simulink model "system"  (R2023a)
settings: Solver=ode15s  StartTime=0.0  StopTime=10.0  MaxStep=1E-3  RelTol=1e-3
libraries: fl_lib x14, nesl_utility x6, slpidlib x1
settings Model: LastModifiedBy=kevin
settings DataIOCC: SaveFormat=Array  ReturnWorkspaceOutputs=off  TimeSaveName=t
settings DebuggingCC: AlgebraicLoopMsg=none  ArtificialAlgebraicLoopMsg=none  MaxConsecutiveZCsMsg=none  ModelReferenceExtraNoncontSigs=none  OperatingPointInterfaceChecksumMismatchMsg=none
settings RTWCC: GPUComputeCapability=5.0

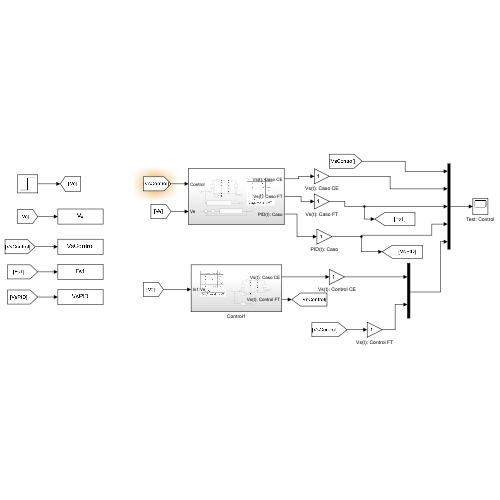
[thumbnail: Simulink's stored preview of the top-level diagram]
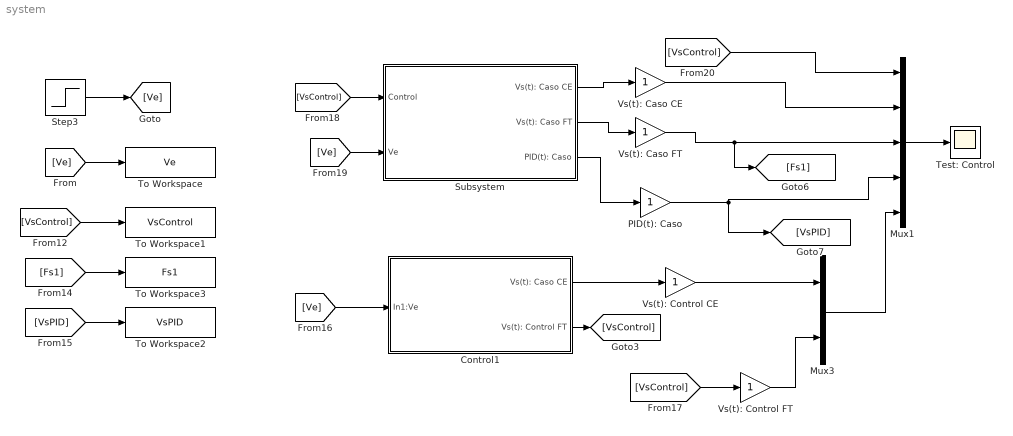
== system system ==
  Control1 : Subsystem
  Mux1 : Mux  Inputs=5
  Mux3 : Mux  Inputs=2
  PID(t): Caso : Gain
  Step3 : Step  Time=0  SampleTime=0
  Subsystem : Subsystem
  Test: Control : Scope
  To Workspace : ToWorkspace  VariableName=Ve  SampleTime=-1
  To Workspace1 : ToWorkspace  VariableName=VsControl  SampleTime=-1
  To Workspace2 : ToWorkspace  VariableName=VsPID  SampleTime=-1
  To Workspace3 : ToWorkspace  VariableName=Fs1  SampleTime=-1
  Vs(t): Caso CE : Gain
  Vs(t): Caso FT : Gain
  Vs(t): Control CE : Gain
  Vs(t): Control FT : Gain
  wires:
  Control1/2(Vs(t): Control FT) -> [VsControl]
  Mux3/1 -> Mux1/5
  Vs(t): Caso CE/1 -> Mux1/2
  Subsystem/3(PID(t): Caso) -> PID(t): Caso/1
  [VsControl] -> Mux1/1
  Mux1/1 -> Test: Control/1
  [Ve] -> Control1/1(In1:Ve)
  [Ve] -> Subsystem/2(Ve)
  [VsControl] -> Subsystem/1(Control)
  Vs(t): Control FT/1 -> Mux3/2
  Subsystem/1(Vs(t): Caso CE) -> Vs(t): Caso CE/1
  PID(t): Caso/1 -> [VsPID], Mux1/4
  [Fs1] -> To Workspace3/1
  [VsControl] -> Vs(t): Control FT/1
  Subsystem/2(Vs(t): Caso FT) -> Vs(t): Caso FT/1
  [VsControl] -> To Workspace1/1
  Control1/1(Vs(t): Caso CE) -> Vs(t): Control CE/1
  Step3/1 -> [Ve]
  Vs(t): Control CE/1 -> Mux3/1
  Vs(t): Caso FT/1 -> [Fs1], Mux1/3
  [Ve] -> To Workspace/1
  [VsPID] -> To Workspace2/1

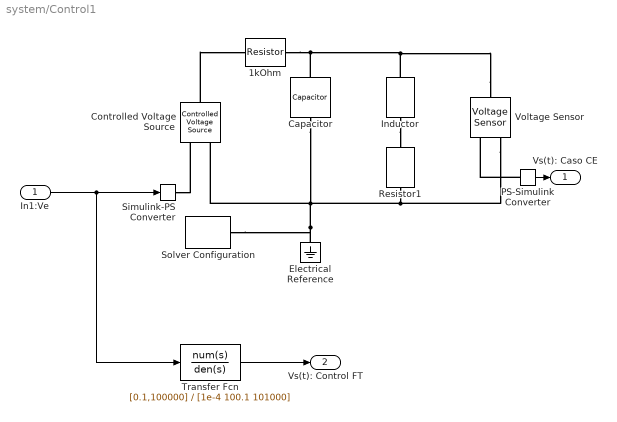
== system system/Control1 ==
  In1:Ve : Inport
  1kOhm : fl_lib/Electrical/Electrical Elements/Resistor  R=1 kOhm  i_specify=off  i_priority=None  i=0 A  i_nominal_specify=off  i_nominal_unit=A  i_nominal_value=1  v_specify=off  v_priority=None  v=0 V  v_nominal_specify=off  v_nominal_unit=V  v_nominal_value=1
  Capacitor : fl_lib/Electrical/Electrical Elements/Capacitor  c=1 uF  r=1e-6 Ohm  g=0 1/Ohm  i_specify=off  i_priority=None  i=0 A  i_nominal_specify=off  i_nominal_unit=A  i_nominal_value=1  v_specify=off  v_priority=None  v=0 V  v_nominal_specify=off  v_nominal_unit=V  v_nominal_value=1  vc_specify=off  vc_priority=High  vc=0 V  vc_nominal_specify=off  vc_nominal_unit=V  vc_nominal_value=1
  Controlled Voltage Source : fl_lib/Electrical/Electrical Sources/Controlled Voltage Source
  Electrical Reference : fl_lib/Electrical/Electrical Elements/Electrical Reference
  Inductor : fl_lib/Electrical/Electrical Elements/Inductor  l=100 mH  r=0 Ohm  g=1e-9 1/Ohm  i_specify=off  i_priority=None  i=0 A  i_nominal_specify=off  i_nominal_unit=A  i_nominal_value=1  v_specify=off  v_priority=None  v=0 V  v_nominal_specify=off  v_nominal_unit=V  v_nominal_value=1  i_L_specify=off  i_L_priority=High  i_L=0 A  i_L_nominal_specify=off  i_L_nominal_unit=A  i_L_nominal_value=1
  PS-Simulink Converter : nesl_utility/PS-Simulink Converter  PhysicalDomain=network_engine_domain  SubClassName=ps_output  LeftPortType=input  RightPortType=output  PseudoPeriodic=off  Frequencies=[]  VectorFormat=inherit  Unit=inherit  AffineConversion=off
  Resistor1 : fl_lib/Electrical/Electrical Elements/Resistor  R=100 kOhm  i_specify=off  i_priority=None  i=0 A  i_nominal_specify=off  i_nominal_unit=A  i_nominal_value=1  v_specify=off  v_priority=None  v=0 V  v_nominal_specify=off  v_nominal_unit=V  v_nominal_value=1
  Simulink-PS Converter : nesl_utility/Simulink-PS Converter  PhysicalDomain=network_engine_domain  SubClassName=ps_input  LeftPortType=input  RightPortType=output  PseudoPeriodic=off  Frequencies=[]  NoiseDistribution=none  NoiseParameters=[]  Unit=1  AffineConversion=off  FilteringAndDerivatives=provide  SimscapeFilterOrder=1  InputFilterTimeConstant=0.001  UdotUserProvided=0
  Solver Configuration : nesl_utility/Solver Configuration  PhysicalDomain=network_engine_domain  SubClassName=solver  LeftPortType=input  RightPortType=generic  Tones=[]  Harmonics=[]  SimulateNoise=off  Profile=off  UseLocalSampling=off  EnableSwitchedLinearOptims=on  FrequencyDomain=off  UseCCode=off  RelTol=0.001  AbsTol=0.001  MinStep=1e-09  ToWorkspace=off  RevertToSquareIcSolve=off  NumHomotopyIterations=100  PhasorMode=off  PhasorModeNumHarmonics=1  ConsistencySolver=NEWTON_XTOL_AFTER_FTOL  IndexReductionMethod=DerivativeReplacement  DoDC=off  ResidualTolerance=1e-09  ConsistencyTolSource=GLOBAL  ConsistencyAbsTol=0.001  ConsistencyRelTol=0.001  ConsistencyTolFactor=0.001  UseLocalSolver=off  LocalSolverChoice=NE_BACKWARD_EULER_ADVANCER  ResolveIndetEquations=on  FunctionEvalNumThread=1  LocalSolverSampleTime=0.001  DoFixedCost=off  MaxNonlinIter=3  MaxModeIter=2  ComputeImpulses=off  ImpulseIterations=2  LinearAlgebra=auto  LinearAlgebraNumThread=0  EquationFormulation=NE_TIME_EF  DelaysMemoryBudget=1024  AutomaticFiltering=on  FilteringTimeConstant=0.001  PartitionStorageMethod=AS_NEEDED  PartitionMemoryBudget=1024  PartitionMethod=ROBUST
  Transfer Fcn : TransferFcn  Numerator=[0.1,100000]  Denominator=[1e-4 100.1 101000]
  Voltage Sensor : fl_lib/Electrical/Electrical Sensors/Voltage Sensor
  Vs(t): Caso CE : Outport
  Vs(t): Control FT : Outport  Port=2
  wires:
  PS-Simulink Converter/1 -> Vs(t): Caso CE/1
  In1:Ve/1 -> Transfer Fcn/1, Simulink-PS Converter/1
  Transfer Fcn/1 -> Vs(t): Control FT/1
  connections:
  Controlled Voltage Source/RConn2 -- Solver Configuration/RConn1 -- Electrical Reference/LConn1 -- Resistor1/LConn1 -- Voltage Sensor/RConn2 -- Capacitor/RConn1
  Voltage Sensor/LConn1 -- 1kOhm/RConn1 -- Capacitor/LConn1 -- Inductor/LConn1
  Inductor/RConn1 -- Resistor1/RConn1
  Simulink-PS Converter/RConn1 -- Controlled Voltage Source/RConn1
  PS-Simulink Converter/LConn1 -- Voltage Sensor/RConn1
  Controlled Voltage Source/LConn1 -- 1kOhm/LConn1

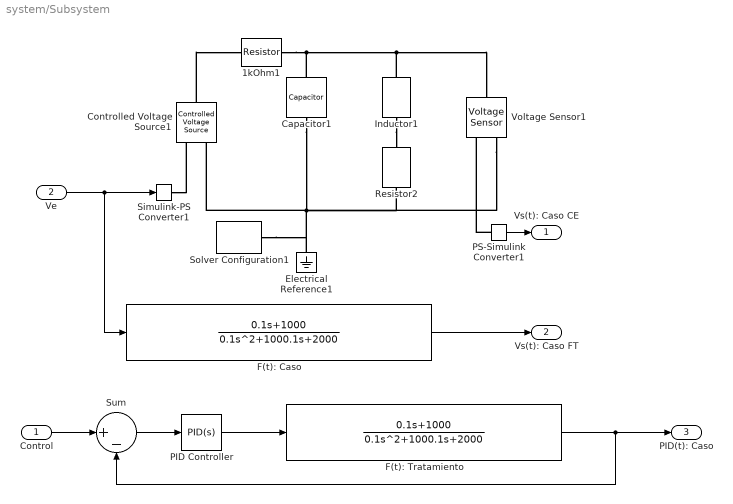
== system system/Subsystem ==
  Control : Inport
  Ve : Inport  Port=2
  1kOhm1 : fl_lib/Electrical/Electrical Elements/Resistor  R=1 kOhm  i_specify=off  i_priority=None  i=0 A  i_nominal_specify=off  i_nominal_unit=A  i_nominal_value=1  v_specify=off  v_priority=None  v=0 V  v_nominal_specify=off  v_nominal_unit=V  v_nominal_value=1
  Capacitor1 : fl_lib/Electrical/Electrical Elements/Capacitor  c=1000 uF  r=1e-6 Ohm  g=0 1/Ohm  i_specify=off  i_priority=None  i=0 A  i_nominal_specify=off  i_nominal_unit=A  i_nominal_value=1  v_specify=off  v_priority=None  v=0 V  v_nominal_specify=off  v_nominal_unit=V  v_nominal_value=1  vc_specify=off  vc_priority=High  vc=0 V  vc_nominal_specify=off  vc_nominal_unit=V  vc_nominal_value=1
  Controlled Voltage Source1 : fl_lib/Electrical/Electrical Sources/Controlled Voltage Source
  Electrical Reference1 : fl_lib/Electrical/Electrical Elements/Electrical Reference
  F(t): Caso : TransferFcn  Numerator=[0.1 1000]  Denominator=[0.1 1000.1 2000]
  F(t): Tratamiento : TransferFcn  Numerator=[0.1 1000]  Denominator=[0.1 1000.1 2000]
  Inductor1 : fl_lib/Electrical/Electrical Elements/Inductor  l=100 mH  r=0 Ohm  g=1e-9 1/Ohm  i_specify=off  i_priority=None  i=0 A  i_nominal_specify=off  i_nominal_unit=A  i_nominal_value=1  v_specify=off  v_priority=None  v=0 V  v_nominal_specify=off  v_nominal_unit=V  v_nominal_value=1  i_L_specify=off  i_L_priority=High  i_L=0 A  i_L_nominal_specify=off  i_L_nominal_unit=A  i_L_nominal_value=1
  PID Controller : slpidlib/PID Controller  Controller=PID  Form=Parallel  TimeDomain=Continuous-time  UseExternalTs=off  SampleTime=-1  IntegratorMethod=Forward Euler  FilterMethod=Forward Euler  ControllerParametersSource=internal  P=400  I=1200  UseKiTs=off  D=0.5  N=2000  UseFilter=on  TunerSelectOption=Transfer Function Based (PID Tuner App)  InitialConditionSource=internal  InitialConditionForIntegrator=0  InitialConditionForFilter=0  DifferentiatorICPrevScaledInput=0  ExternalReset=none  TrackingMode=off  Kt=1  LimitOutput=off  SatLimitsSource=internal  UpperSaturationLimit=inf  LowerSaturationLimit=-inf  LinearizeAsGain=on  AntiWindupMode=none  Kb=1  LimitIntegrator=off  UpperIntegratorSaturationLimit=inf  LowerIntegratorSaturationLimit=-inf  POutMin=[]  POutMax=[]  IOutMin=[]  IOutMax=[]  DOutMin=[]  DOutMax=[]  NOutMin=[]  NOutMax=[]  SumOutMin=[]  SumOutMax=[]  SaturationOutMin=[]  SaturationOutMax=[]  PParamMin=[]  PParamMax=[]  IParamMin=[]  IParamMax=[]  DParamMin=[]  DParamMax=[]  NParamMin=[]  NParamMax=[]  KbParamMin=[]  KbParamMax=[]  KtParamMin=[]  KtParamMax=[]  KbOutMin=[]  KbOutMax=[]  KtOutMin=[]  KtOutMax=[]  IntegratorOutMin=[]  IntegratorOutMax=[]  FilterOutMin=[]  FilterOutMax=[]  SumI1OutMin=[]  SumI1OutMax=[]  SumI2OutMin=[]  SumI2OutMax=[]  SumI3OutMin=[]  SumI3OutMax=[]  SumI4OutMin=[]  SumI4OutMax=[]  SumDOutMin=[]  SumDOutMax=[]  DifferentiatorOutMin=[]  DifferentiatorOutMax=[]  FilterDiffOutCoefMin=[]  FilterDiffOutCoefMax=[]  ReciprocalOutMin=[]  ReciprocalOutMax=[]  SumDenOutMin=[]  SumDenOutMax=[]  SumNumOutMin=[]  SumNumOutMax=[]  DivideOutMin=[]  DivideOutMax=[]  UdiffTsProdOutMin=[]  UdiffTsProdOutMax=[]  NTsProdOutMin=[]  NTsProdOutMax=[]  UintegralTsProdOutMin=[]  UintegralTsProdOutMax=[]  UngainTsProdOutMin=[]  UngainTsProdOutMax=[]  ClampingZeroOutDataTypeStr=Inherit: Inherit via back propagation  ClampingZeroOutMin=[]  ClampingZeroOutMax=[]  FilterDenConstantOutDataTypeStr=Inherit: Inherit via back propagation  FilterDenConstantOutMin=[]  FilterDenConstantOutMax=[]  PCopyOutDataTypeStr=Inherit: Inherit via back propagation  PCopyOutMin=[]  PCopyOutMax=[]  NCopyOutDataTypeStr=Inherit: Inherit via back propagation  NCopyOutMin=[]  NCopyOutMax=[]  IntegratorContinuousStateAttributes=''  IntegratorStateMustResolveToSignalObject=off  IntegratorRTWStateStorageClass=Auto  FilterContinuousStateAttributes=''  FilterStateMustResolveToSignalObject=off  FilterRTWStateStorageClass=Auto  ParallelPVariant=InternalParameters  IdealPVariant=Disabled  IVariant=InternalParameters  DVariant=InternalParameters  IntegratorVariant=Continuous  SatVariant=Disabled  AWVariant=Passthrough  PCopyVariant=Disabled  TRVariant=Disabled  FdbkBlocksVariant=Forward  IdealPFdbkVariant=Disabled  SatFdbkVariant=Disabled  DerivativeFilterVariant=ContFilter  NVariant=InternalParameters  NCopyVariant=Disabled  FilterICVariant=InternalICsFilter  IntegratorICVariant=InternalICs  ExternalResetVariant=Disabled  TRSumVariant=Passthrough  SumFdbkVariant=Disabled  SumVariant=Sum_PID  TsampFilterVariant=InternalTs  TsampNgainVariant=Passthrough  TsampIntegralVariant=Disabled_SignalSpec  ExternalSaturationOutDataTypeStr=Inherit: Same as second input
  PS-Simulink Converter1 : nesl_utility/PS-Simulink Converter  PhysicalDomain=network_engine_domain  SubClassName=ps_output  LeftPortType=input  RightPortType=output  PseudoPeriodic=off  Frequencies=[]  VectorFormat=inherit  Unit=inherit  AffineConversion=off
  Resistor2 : fl_lib/Electrical/Electrical Elements/Resistor  R=1 kOhm  i_specify=off  i_priority=None  i=0 A  i_nominal_specify=off  i_nominal_unit=A  i_nominal_value=1  v_specify=off  v_priority=None  v=0 V  v_nominal_specify=off  v_nominal_unit=V  v_nominal_value=1
  Simulink-PS Converter1 : nesl_utility/Simulink-PS Converter  PhysicalDomain=network_engine_domain  SubClassName=ps_input  LeftPortType=input  RightPortType=output  PseudoPeriodic=off  Frequencies=[]  NoiseDistribution=none  NoiseParameters=[]  Unit=1  AffineConversion=off  FilteringAndDerivatives=provide  SimscapeFilterOrder=1  InputFilterTimeConstant=0.001  UdotUserProvided=0
  Solver Configuration1 : nesl_utility/Solver Configuration  PhysicalDomain=network_engine_domain  SubClassName=solver  LeftPortType=input  RightPortType=generic  Tones=[]  Harmonics=[]  SimulateNoise=off  Profile=off  UseLocalSampling=off  EnableSwitchedLinearOptims=on  FrequencyDomain=off  UseCCode=off  RelTol=0.001  AbsTol=0.001  MinStep=1e-09  ToWorkspace=off  RevertToSquareIcSolve=off  NumHomotopyIterations=100  PhasorMode=off  PhasorModeNumHarmonics=1  ConsistencySolver=NEWTON_XTOL_AFTER_FTOL  IndexReductionMethod=DerivativeReplacement  DoDC=off  ResidualTolerance=1e-09  ConsistencyTolSource=GLOBAL  ConsistencyAbsTol=0.001  ConsistencyRelTol=0.001  ConsistencyTolFactor=0.001  UseLocalSolver=off  LocalSolverChoice=NE_BACKWARD_EULER_ADVANCER  ResolveIndetEquations=on  FunctionEvalNumThread=1  LocalSolverSampleTime=0.001  DoFixedCost=off  MaxNonlinIter=3  MaxModeIter=2  ComputeImpulses=off  ImpulseIterations=2  LinearAlgebra=auto  LinearAlgebraNumThread=0  EquationFormulation=NE_TIME_EF  DelaysMemoryBudget=1024  AutomaticFiltering=on  FilteringTimeConstant=0.001  PartitionStorageMethod=AS_NEEDED  PartitionMemoryBudget=1024  PartitionMethod=ROBUST
  Sum : Sum  Inputs=|+-
  Voltage Sensor1 : fl_lib/Electrical/Electrical Sensors/Voltage Sensor
  Vs(t): Caso CE : Outport
  Vs(t): Caso FT : Outport  Port=2
  PID(t): Caso : Outport  Port=3
  wires:
  Ve/1 -> F(t): Caso/1, Simulink-PS Converter1/1
  PS-Simulink Converter1/1 -> Vs(t): Caso CE/1
  F(t): Caso/1 -> Vs(t): Caso FT/1
  PID Controller/1 -> F(t): Tratamiento/1
  Control/1 -> Sum/1
  Sum/1 -> PID Controller/1
  F(t): Tratamiento/1 -> PID(t): Caso/1, Sum/2
  connections:
  Capacitor1/RConn1 -- Solver Configuration1/RConn1 -- Electrical Reference1/LConn1 -- Resistor2/LConn1 -- Voltage Sensor1/RConn2 -- Controlled Voltage Source1/RConn2
  Capacitor1/LConn1 -- Voltage Sensor1/LConn1 -- Inductor1/LConn1 -- 1kOhm1/RConn1
  Simulink-PS Converter1/RConn1 -- Controlled Voltage Source1/RConn1
  PS-Simulink Converter1/LConn1 -- Voltage Sensor1/RConn1
  Controlled Voltage Source1/LConn1 -- 1kOhm1/LConn1
  Inductor1/RConn1 -- Resistor2/RConn1
